simulink model "ProbeStateFlow"  (R2025b)
settings: Solver=FixedStepDiscrete  StartTime=0.0  StopTime=inf  FixedStep=0.1  RelTol=1e-3
model workspace (MAT data in the model file):
  Coupling = Simulink.Signal
  Coupling.Dimensions = 1
  Coupling.DimensionsMode = 'Fixed'
  Coupling.Complexity = 'real'
  Coupling.SampleTime = -1
  Coupling.SamplingMode = 'auto'
  Coupling.InitialValue = '0'
  Coupling.DataType = 'uint8'
  DAC1_ch2 = Simulink.Signal
  DAC1_ch2.Dimensions = 1
  DAC1_ch2.DimensionsMode = 'Fixed'
  DAC1_ch2.Complexity = 'real'
  DAC1_ch2.SampleTime = -1
  DAC1_ch2.SamplingMode = 'auto'
  DAC1_ch2.DataType = 'uint16'
  D_FallingEdgePos = Simulink.Signal
  D_FallingEdgePos.Dimensions = 1
  D_FallingEdgePos.DimensionsMode = 'Fixed'
  D_FallingEdgePos.Complexity = 'real'
  D_FallingEdgePos.SampleTime = -1
  D_FallingEdgePos.SamplingMode = 'auto'
  D_FallingEdgePos.InitialValue = '0'
  D_FallingEdgePos.DataType = 'uint32'
  GeneratorChannel = Simulink.Signal
  GeneratorChannel.Dimensions = 1
  GeneratorChannel.DimensionsMode = 'Fixed'
  GeneratorChannel.Complexity = 'real'
  GeneratorChannel.SampleTime = -1
  GeneratorChannel.SamplingMode = 'auto'
  GeneratorChannel.InitialValue = '0'
  GeneratorChannel.DataType = 'uint8'
  IsDualProbe = Simulink.Signal
  IsDualProbe.Dimensions = 1
  IsDualProbe.DimensionsMode = 'Fixed'
  IsDualProbe.Complexity = 'real'
  IsDualProbe.SampleTime = -1
  IsDualProbe.SamplingMode = 'auto'
  IsDualProbe.InitialValue = '1'
  IsDualProbe.DataType = 'uint8'
  PE_BlueZero = Simulink.Signal
  PE_BlueZero.Dimensions = 1
  PE_BlueZero.DimensionsMode = 'Fixed'
  PE_BlueZero.Complexity = 'real'
  PE_BlueZero.SampleTime = -1
  PE_BlueZero.SamplingMode = 'auto'
  PE_BlueZero.DataType = 'uint16'
  PE_RedZero = Simulink.Signal
  PE_RedZero.Dimensions = 1
  PE_RedZero.DimensionsMode = 'Fixed'
  PE_RedZero.Complexity = 'real'
  PE_RedZero.SampleTime = -1
  PE_RedZero.SamplingMode = 'auto'
  PE_RedZero.DataType = 'uint16'
  PE_Settings = Simulink.Signal
  PE_Settings.Dimensions = 1
  PE_Settings.DimensionsMode = 'Fixed'
  PE_Settings.Complexity = 'real'
  PE_Settings.SampleTime = -1
  PE_Settings.SamplingMode = 'auto'
  PE_Settings.InitialValue = 'PE_SettingsInitStruct'
  PE_Settings.DataType = 'Bus: tPE_Settings'
  PE_ZeroCurrent = Simulink.Signal
  PE_ZeroCurrent.Dimensions = 1
  PE_ZeroCurrent.DimensionsMode = 'Fixed'
  PE_ZeroCurrent.Complexity = 'real'
  PE_ZeroCurrent.SampleTime = -1
  PE_ZeroCurrent.SamplingMode = 'auto'
  PE_ZeroCurrent.DataType = 'uint16'
  PE_ZeroFiltered = Simulink.Signal
  PE_ZeroFiltered.Dimensions = 1
  PE_ZeroFiltered.DimensionsMode = 'Fixed'
  PE_ZeroFiltered.Complexity = 'real'
  PE_ZeroFiltered.SampleTime = -1
  PE_ZeroFiltered.SamplingMode = 'auto'
  PE_ZeroFiltered.DataType = 'uint16'
  ProbeType = Simulink.Signal
  ProbeType.Dimensions = 1
  ProbeType.DimensionsMode = 'Fixed'
  ProbeType.Complexity = 'real'
  ProbeType.SampleTime = -1
  ProbeType.SamplingMode = 'auto'
  ProbeType.InitialValue = '0'
  ProbeType.DataType = 'uint8'
  Signal = Simulink.Signal
  Signal.Dimensions = 19944
  Signal.DimensionsMode = 'Fixed'
  Signal.Complexity = 'real'
  Signal.SampleTime = -1
  Signal.SamplingMode = 'auto'
  Signal.InitialValue = 'ones(1, 19944)*1975'
  Signal.DataType = 'uint16'
  SignalDC = Simulink.Signal
  SignalDC.Dimensions = 1
  SignalDC.DimensionsMode = 'Fixed'
  SignalDC.Complexity = 'real'
  SignalDC.SampleTime = -1
  SignalDC.SamplingMode = 'auto'
  SignalDC.InitialValue = '0'
  SignalDC.DataType = 'uint16'
  SingleDual = Simulink.Signal
  SingleDual.Dimensions = 1
  SingleDual.DimensionsMode = 'Fixed'
  SingleDual.Complexity = 'real'
  SingleDual.SampleTime = -1
  SingleDual.SamplingMode = 'auto'
  SingleDual.InitialValue = '0'
  SingleDual.DataType = 'uint8'
  ZondB_Width = Simulink.Signal
  ZondB_Width.Dimensions = 1
  ZondB_Width.DimensionsMode = 'Fixed'
  ZondB_Width.Complexity = 'real'
  ZondB_Width.SampleTime = -1
  ZondB_Width.SamplingMode = 'auto'
  ZondB_Width.InitialValue = '0'
  ZondB_Width.DataType = 'uint8'
settings Model: DataDictionary=ProbeStateFlow_Data.sldd  Creator=lolve  LastModifiedBy=lolve
settings OptimizationCC: UseDivisionForNetSlopeComputation=on  GainParamInheritBuiltInType=on  UseFloatMulNetSlope=on  OptimizeBlockIOStorage=off  BufferReuse=off  ReuseModelBlockBuffer=off  GlobalBufferReuse=off  ExpressionFolding=off  EnableMemcpy=off  PassReuseOutputArgsAs=Individual arguments  LocalBlockOutputs=off  ZeroExternalMemoryAtStartup=off  ZeroInternalMemoryAtStartup=off  NoFixptDivByZeroProtection=on  EfficientFloat2IntCast=on  LifeSpan=1  OptimizeDataStoreBuffers=off  BusAssignmentInplaceUpdate=off  OptimizationLevel=level0  OptimizationCustomize=off  EfficientTunableParamExpr=on
settings DebuggingCC: SignalResolutionControl=None  ParameterTunabilityLossMsg=error
settings HardwareCC: ProdLongLongMode=on
settings SFSimCC: MATLABDynamicMemAlloc=off
settings RTWCC: SystemTargetFile=ert.tlc  GenCodeOnly=on  TemplateMakefile=ert_default_tmf  GenerateReport=on  LaunchReport=on  Description=Embedded Coder
settings CodeAppCC: ForceParamTrailComments=on  IgnoreCustomStorageClasses=off  OperatorAnnotations=on  SimulinkDataObjDesc=on  SFDataObjDesc=on  CustomSymbolStrGlobalVar=rt$N$M  CustomSymbolStrType=$N$M  CustomSymbolStrFcn=$N$M$F  CustomSymbolStrMacro=$N$M  InsertBlockDesc=on  StateflowObjectComments=on  MATLABSourceComments=on
settings ERTTargetCC: InlinedParameterPlacement=Hierarchical  ERTCustomFileTemplate=example_file_process.tlc  ERTFilePackagingFormat=CompactWithDataFile  TargetLangStandard=C99 (ISO)  GenerateSampleERTMain=on  IncludeMdlTerminateFcn=off  CombineSignalStateStructs=on  SupportAbsoluteTime=off  SupportComplex=off  SupportNonInlinedSFcns=on

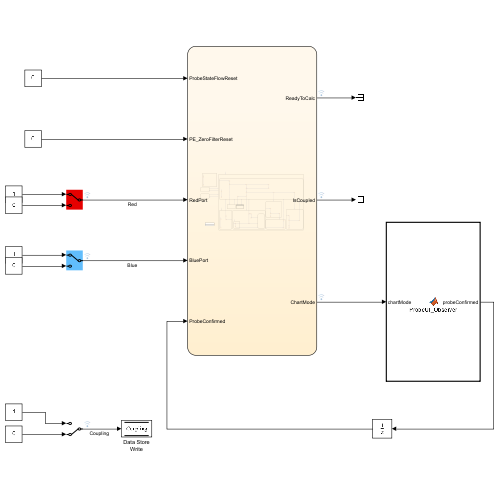
[thumbnail: Simulink's stored preview of the top-level diagram]
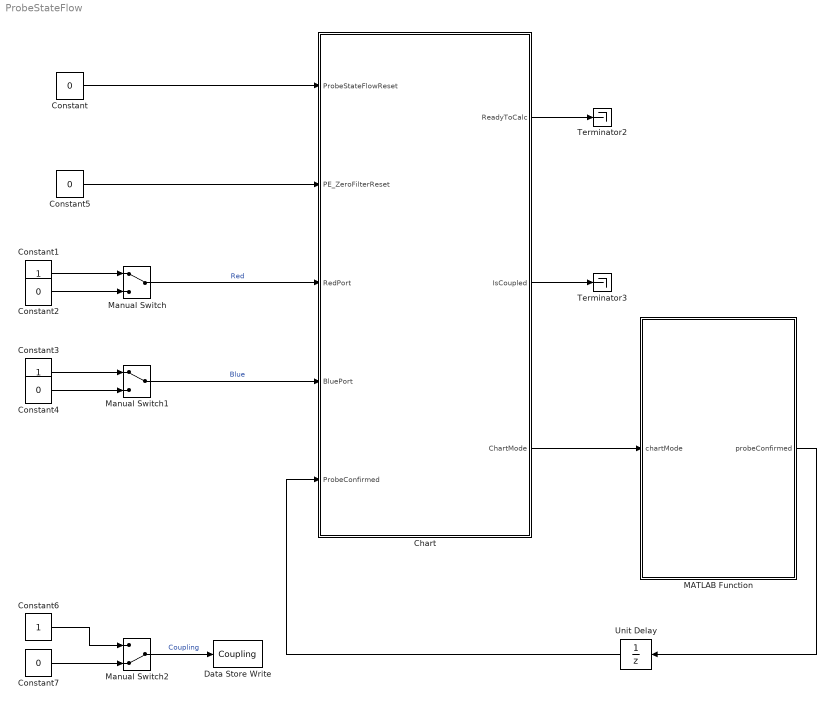
== system ProbeStateFlow ==
  Chart : Stateflow chart  TreatAsAtomicUnit=on
      settings: PortSchema="{\"entries\":[{\"content\":{\"sides\":[{\"content\":{\"connectorIds\":[\"In1\",\"In4\",\"In2\",\"In3\",\"In5\"]},\"type\":\"ConnectorPlacement.EquallySpacedRectSide\",\"uuid\":\"9a633d17-6e12-4111-a0d1-d38bdd533965\"},{\"content\":{\"connectorIds\":[\"Out2\",\"Out3\",\"Out1\"],\"side\":\"RIGHT\"},\"type\":\"ConnectorPlacement.EquallySpacedRectSide\",\"uuid\":\"ec8af492-d901-445a-be79-664e940aa17f\"},{\"content\":{\"side\":\"TOP\"},\"type\":\"ConnectorPlacement.EquallySpacedRectSide\",\"uuid\":\"56b2aa18-34f3-4c88-8d68-b210a846aede\"}]},\"type\":\"ConnectorPlacement.EquallySpacedConnector\",\"uuid\":\"7e595df7-d9a5-4a82-bd1b-a8dba317762f\"}],\"packageUris\":[\"http://schema.mathworks.com/mf0/Connector/R2020b\"],\"version\":\"1.0\"}"
  Constant{,2,4..5} (4 alike) : Constant  Value=0
  Constant1 : Constant
  Constant3 : Constant
  Constant6 : Constant  OutDataTypeStr=uint8
  Constant7 : Constant  Value=0  OutDataTypeStr=uint8
  Data Store Write : DataStoreWrite  DataStoreName=Coupling  DataStoreElements=Coupling  IndexOptions=Index vector (dialog)  Indices=1  OutputSizes=1
  MATLAB Function : MATLAB Function  TreatAsAtomicUnit=on
      settings: RTWSystemCode=Inline
  Manual Switch : ManualSwitch
  Manual Switch1 : ManualSwitch
  Manual Switch2 : ManualSwitch  CurrentSetting=0
  Terminator2 : Terminator
  Terminator3 : Terminator
  Unit Delay : UnitDelay  SampleTime=-1  HasFrameUpgradeWarning=on
  wires:
  Chart/1(ChartMode) -> MATLAB Function/1(chartMode)
  Constant/1 -> Chart/1(ProbeStateFlowReset)
  Constant1/1 -> Manual Switch/1
  Constant2/1 -> Manual Switch/2
  Manual Switch/1 -> Chart/2(RedPort)  "Red"
  Constant3/1 -> Manual Switch1/1
  Constant4/1 -> Manual Switch1/2
  Manual Switch1/1 -> Chart/3(BluePort)  "Blue"
  Constant5/1 -> Chart/4(PE_ZeroFilterReset)
  Constant7/1 -> Manual Switch2/2
  Constant6/1 -> Manual Switch2/1
  Manual Switch2/1 -> Data Store Write/1  "Coupling"
  Chart/2(ReadyToCalc) -> Terminator2/1
  Chart/3(IsCoupled) -> Terminator3/1
  MATLAB Function/1(probeConfirmed) -> Unit Delay/1
  Unit Delay/1 -> Chart/5(ProbeConfirmed)

== matlab function ProbeStateFlow/MATLAB Function ==
  data: chartMode input; probeConfirmed output
function probeConfirmed = ProbeUI_Observer(chartMode)
    %#codegen
    coder.extrinsic('updateProbeUI');
    
    probeConfirmed = uint8(0);
    
    % Условие 1: немодальный список совмещенных ПЭП
    isWaitingSingle = (chartMode == ChartModeType.WaitProbeSelect);
    
    % Условие 2: модальное подтверждение Р/С ПЭП при входе в PE_ZeroGainAdjust
    isZeroAdjust = (chartMode == ChartModeType.PE_ZeroGainAdjust);
    
    [probeConfirmed, ~] = updateProbeUI(isWaitingSingle, isZeroAdjust);
end

== stateflow chart ProbeStateFlow/Chart ==
  state ProbeStateFlow
    entry, during:
    Do(tAction.RemoveDC);
    state CheckConnectionRed
      CheckConnectionRed -> (junction 183)
      (junction 183) -> (junction 51) : {IsProbeRedConnected = Do(tAction.CheckConnection);}
      (junction 51) -> (junction 56) [order 1] : [IsProbeRedConnected]
      (junction 56) -> (junction 59) [order 1] : [IsProbeBlueConnected || IsDualProbe == 0]
      (junction 56) -> (junction 71) [order 2]
      (junction 59) -> (junction 61) : {IsProbeConnected = 1;}
      (default) -> (junction 205)
      (junction 205) -> (junction 207) : {SingleDual = 0;
          | ZondB_Width = 5;
          | GeneratorChannel = 0;
          | Do(tAction.DAC1_BufFill,...
          | uint32( 10));}
      (junction 61) -> (junction 71)
      (junction 71) -> (junction 63)
      (junction 63) -> (junction 65) [order 1] : [WasProbeConnected]
      (junction 65) -> (junction 160) [order 1] : [MeasureMethod == EE || IsDualProbe == 0]
      (junction 63) -> (junction 67) [order 2]
      (junction 67) -> (junction 69) [order 1] : [IsProbeConnected]
    state PrepareToPE
      entry:
      SingleDual = 1;
      ZondB_Width = 5;
      Do(tAction.GainCurveBufFill);
      D_FallingEdgePos = uint32(PE_Settings.Dpos);
      DAC1_ch2 = PE_Settings.Threshold;
      PrepareToPE -> (junction 167)
      (junction 167) -> (junction 281) : {DAC1_ch2 = PE_Settings.Threshold;
          | IsCoupled = Do(tAction.CouplingCheckPE);
          | ReadyToCalc = IsCoupled;}
      (junction 281) -> (junction 171) [order 1] : [IsCoupled == 0]
      (junction 281) -> (junction 372) [order 2]
    state PrepareToEE
      entry:
      IsReadyToMeasure = 1;
      ZondB_Width = 5;
      SingleDual = IsDualProbe;
      %StaticGainBufFill(147);
      Do(tAction.StaticGainBufFill);
      PrepareToEE -> (junction 287)
      (junction 287) -> (junction 289) : {IsCoupled =...
          |   Do(tAction.CouplingCheckEE);}
      (junction 289) -> (junction 294) [order 1] : [IsCoupled == 0]
      (junction 289) -> (junction 299) [order 2] : {IsGainAdjusting = Do(tAction.GainAdjust);
          | %StaticGainBufFill(147);
          | Do(tAction.StaticGainBufFill);
          | ReadyToCalc = ...
          |  uint16(~IsGainAdjusting);}
      (junction 299) -> (junction 328)
    state RedDisconnect
      entry:
      ResetFlags
    state GetProbeProperties
      state ProbeParamsStart
        ProbeParamsStart -> (junction 105)
      state ProbeParamsFinish
        during:
        WasProbeConnected = 1;
      state DelayLine
        DelayLine -> (junction 112)
      state CouplingSNR
        (default) -> (junction 251)
        (junction 251) -> (junction 253) : {SingleDual = 1;}
        CouplingSNR -> (junction 120)
        (junction 120) -> (junction 240)
      state PE_ZeroGainAdjust
        entry:
        ZondB_Width = PE_Settings.ZeroZondWidth;
        SingleDual = 0;
      state PE_BlueZeroMeasure
        entry:
        GeneratorChannel = 1;
        PE_BlueZeroMeasure -> (junction 377)
        (junction 377) -> (junction 380) : {PE_BlueZero = Do(tAction.PE_ZeroCalc);}
        (junction 380) -> (junction 383)
      (default) -> ProbeParamsStart
      (junction 105) -> ProbeParamsFinish
      ProbeParamsFinish -> DelayLine : [WasProbeConnected]
      (junction 112) -> CouplingSNR
      (junction 240) -> (junction 237) [order 1] : [IsDualProbe == 0]
      (junction 240) -> PE_ZeroGainAdjust [order 2]
      (junction 383) -> (junction 237)
      PE_ZeroGainAdjust -> PE_BlueZeroMeasure
    state CalcDC
      (junction 48) -> (junction 218) : {SignalDC =...
          |  Do(tAction.CalcDC);}
      (default) -> (junction 212)
      CalcDC -> (junction 48)
      (junction 212) -> (junction 214) : {SingleDual = 0;
          | ZondB_Width = 0;
          | GeneratorChannel = 0;
          | Do(tAction.DAC1_BufFill);}
    state CheckConnectionBlue
      entry:
      SingleDual = 1;
      ZondB_Width = 5;
      GeneratorChannel = 1;
      Do(tAction.DAC1_BufFill);
      during:
      IsProbeBlueConnected =...
      Do(tAction.CheckConnection);
      state WaitProbeSelect
      state CheckBlue
        CheckBlue -> (junction 365)
        (junction 365) -> (junction 367) [order 2] : {ResetFlags;}
      (junction 360) -> (junction 357)
      (junction 353) -> (junction 357) : {IsDualProbe = 1;}
      (junction 358) -> (junction 360) : {IsDualProbe = 0;}
      WaitProbeSelect -> (junction 358) [order 2] : [ProbeConfirmed]
      (default) -> CheckBlue
      (junction 365) -> (junction 353) [order 1] : [IsProbeBlueConnected]
      WaitProbeSelect -> (junction 353) [order 1] : [IsProbeBlueConnected]
      (junction 367) -> WaitProbeSelect
    state PE_zero
      entry:
      ZondB_Width = 5;
      SingleDual = 0;
      %StaticGainBufFill(GainForPE_Zero_DAC);
      Do(tAction.StaticGainBufFill);
      (junction 275) -> (junction 277) : {PE_ZeroCurrent = Do(tAction.PE_ZeroCalc);
          | PE_ZeroFiltered = Do(tAction.PE_ZeroFilter);
          | IsReadyToMeasure = 1;}
      PE_zero -> (junction 275)
    (junction 51) -> RedDisconnect [order 2] : after(1, sec)
    (junction 65) -> PrepareToPE [order 2]
    (junction 160) -> PrepareToEE
    (junction 69) -> GetProbeProperties
    (junction 67) -> CheckConnectionBlue [order 2]
    (junction 218) -> CheckConnectionRed
    RedDisconnect -> CheckConnectionRed
    (junction 357) -> CheckConnectionRed
    (junction 277) -> CheckConnectionRed
    (junction 294) -> CheckConnectionRed : {ReadyToCalc = 0;
        | Do(tAction.GainAdjustReset);}
    (default) -> CalcDC
    (junction 171) -> PE_zero
    (junction 237) -> CheckConnectionRed
  state ResetState
    entry:
    ResetFlags
  state PE_ZeroFilterResetState
    entry:
    IsPE_ZeroBuffFilled = 0;
    PE_ZeroBufIdx = 0;
  state ResetFlags [function]
    (default) -> (junction 262)
    (junction 262) -> (junction 265) : {IsProbeConnected = 0;
        | WasProbeConnected = 0;
        | IsProbeBlueConnected = 0;
        | IsDualProbe = 1;
        | IsReadyToMeasure = 0;
        | IsPE_ZeroBuffFilled = 0;
        | PE_ZeroBufIdx = 0;
        | Do(tAction.GainAdjustReset);}
  (default) -> ProbeStateFlow
  ResetState -> ProbeStateFlow
  ProbeStateFlow -> ResetState [order 1] : [ProbeStateFlowReset]
  PE_ZeroFilterResetState -> ProbeStateFlow
  ProbeStateFlow -> PE_ZeroFilterResetState [order 2] : [PE_ZeroFilterReset]
  data: action function_input Enum: tAction size=1; res function_output uint16 size=1; varargin function_input; ChartMode output Enum: ChartModeType; WasProbeConnected local =0; IsProbeConnected local =0; EE constant double =0; MeasureMethod local =1; ProbeStateFlowReset input; RedPort input; BluePort input; SingleDual data_store_memory; ZondB_Width data_store_memory; GeneratorChannel data_store_memory; SignalDC data_store_memory; IsDualProbe data_store_memory =0; IsPE_ZeroBuffFilled local =0; IsReadyToMeasure local =0; PE_ZeroBufIdx local =0; PE_ZeroFilterReset input; GainForPE_Zero_DAC local =116; Coupling data_store_memory; IsGainAdjusting local uint16 size=1 =0; ReadyToCalc output uint16 size=1 =0; IsCoupled output uint16 size=1 =0; ProbeConfirmed input size=1; PE_Settings data_store_memory; Signal data_store_memory size=19944; IsProbeRedConnected local uint16 size=1 =0; IsProbeBlueConnected local uint16 size=1 =0; DAC1_ch2 data_store_memory; D_FallingEdgePos data_store_memory; PE_ZeroCurrent data_store_memory; PE_ZeroFiltered data_store_memory; PE_BlueZero data_store_memory
  function res = Do(action, varargin):
    | function res = Do(action, varargin)
    | %#codegen
    | coder.inline('always');
    | res = uint16(0);
    | 
    | arg1 = int32(0); arg2 = int32(0); arg3 = int32(0);
    | if numel(varargin) >= 1, arg1 = int32(varargin{1}); end
    | if numel(varargin) >= 2, arg2 = int32(varargin{2}); end
    | if numel(varargin) >= 3, arg3 = int32(varargin{3}); end
    | 
    | if coder.target('Rtw')
    |     % При генерации кода под STM32 вызывается единая Си-функция с 4 аргументами
    |     res = coder.ceval('Do', action, arg1, arg2, arg3);
    | else
    | 
    |     switch action
    |         case tAction.CalcDC
    |             res = uint16( 1975);
    |         case tAction.CheckConnection
    |             if SingleDual == 0
    |                 res = uint16( RedPort);
    |             else
    |                 res = uint16( BluePort);
    |             end
    |         case tAction.RemoveDC
    |             res = uint16(0);
    |         case tAction.CouplingCheckPE
    |             res = uint16( Coupling);
    |         case tAction.CouplingCheckEE
    |             res = uint16( Coupling);
    |         case tAction.GainAdjustReset
    |             res = uint16(0);
    |         case tAction.GainCurveBufFill
    |             res = uint16(0);
    |         case tAction.DAC1_BufFill
    |             res = uint16(arg1);
    |         case tAction.StaticGainBufFill
    |             res = uint16(0);
    |         case tAction.PE_ZeroCalc
    |             res = uint16(0);
    |         case tAction.PE_ZeroFilter
    |             res = uint16(0);
    |     end
    | end
